simulink model "pdoublet_lin"  (R2025a)
settings: Solver=VariableStepAuto  StartTime=0.0  StopTime=20  FixedStep=0.005  RelTol=1e-3
undefined symbols (not defined in the file): A, B, C, D, K, T
settings Model: Creator=guima  LastModifiedBy=guima
settings SolverCC: AlgebraicLoopSolver=TrustRegion
settings DataIOCC: ReturnWorkspaceOutputs=off
settings DebuggingCC: UnconnectedInputMsg=warning  UnconnectedOutputMsg=warning  UnconnectedLineMsg=warning
settings ModelReferenceCC: EnableRefExpFcnMdlSchedulingChecks=on
settings RTWCC: GPUComputeCapability=3.5

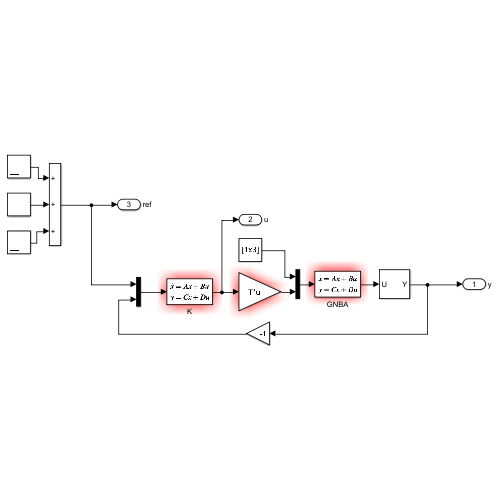
[thumbnail: Simulink's stored preview of the top-level diagram]
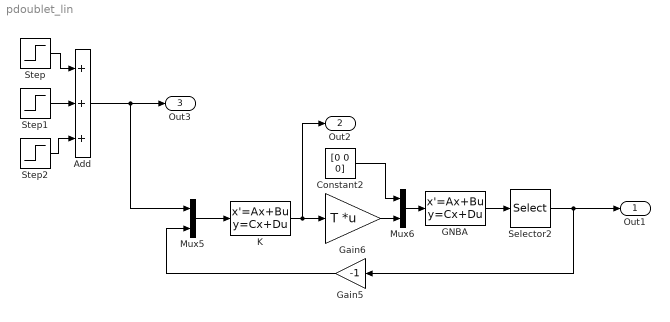
== system pdoublet_lin ==
  Add : Sum  Inputs=+++
  Constant2 : Constant  Value=[0 0 0]
  GNBA : StateSpace  A=A  B=B  C=C  D=D  InitialCondition=0
  Gain5 : Gain  Gain=-1
  Gain6 : Gain  Gain=T  Multiplication=Matrix(K*u)
  K : StateSpace  A=K.A  B=K.B  C=K.C  D=K.D  InitialCondition=0
  Mux5 : Mux  Inputs=2
  Mux6 : Mux  Inputs=2
  Selector2 : Selector  InputPortWidth=1681  IndexOptions=Index vector (dialog)  Indices=[1680,1681,1630,1627]  OutputSizes=1
  Step : Step  Time=5  SampleTime=0
  Step1 : Step  Time=10  After=-2  SampleTime=0
  Step2 : Step  Time=15  SampleTime=0
  Out1 : Outport  SignalName=y
  Out2 : Outport  Port=2  SignalName=u
  Out3 : Outport  Port=3  SignalName=ref
  wires:
  Step1/1 -> Add/2
  Step2/1 -> Add/3
  Step/1 -> Add/1
  Selector2/1 -> Out1/1, Gain5/1
  Gain5/1 -> Mux5/2
  Gain6/1 -> Mux6/2
  Mux5/1 -> K/1
  GNBA/1 -> Selector2/1
  Constant2/1 -> Mux6/1
  Mux6/1 -> GNBA/1
  K/1 -> Out2/1, Gain6/1
  Add/1 -> Out3/1, Mux5/1
